simulink model "FOCsimulation"  (R2023b)
settings: Solver=VariableStepAuto  StartTime=0.0  StopTime=12  RelTol=1e-3
values from neighbouring files (symbols this model uses):
  acceleration = 20000/PU_System.N_base    [FOC_Script.m]    (also in Motor_script.m)
  PI_params = mcb.internal.SetControllerParameters(pmsm,inverter,PU_System,T_pwm,2*Ts,Ts_speed)    [FOC_Script.m]    (also in Motor_script.m)
  Speed_openLoop_PU = 0.1    [FOC_Script.m]    (also in Motor_script.m)
  T_Ref_openLoop = 1    [FOC_Script.m]    (also in Motor_script.m)
  Ts = T_pwm    (= 0.0001)    [FOC_Script.m]    (also in Motor_script.m = 3.33333333333e-05)
  Ts_motor = T_pwm/2    (= 5e-05)    [FOC_Script.m]    (also in Motor_script.m = 1.66666666667e-05)
  Ts_speed = 30*Ts    (= 0.003)    [FOC_Script.m]    (also in Motor_script.m = 0.001)
undefined symbols (not defined in the file or in its folder): inverter, pmsm, PU_System, sigbuilder_block, target
libraries: mcbcontrolslib x11, slpidlib x3, mcbpositiondecoderlib x2, simulink x1, dspsrcs4 x1, mcbplantlib x1, autolibpmsmexterior x1
(part 1 of 2)
settings Model: Creator=Juan Camilo  LastModifiedBy=84339
settings DebuggingCC: UnconnectedInputMsg=warning  UnconnectedOutputMsg=warning  UnconnectedLineMsg=warning
settings ModelReferenceCC: EnableRefExpFcnMdlSchedulingChecks=on
settings RTWCC: DLArmComputeVersion=19.05

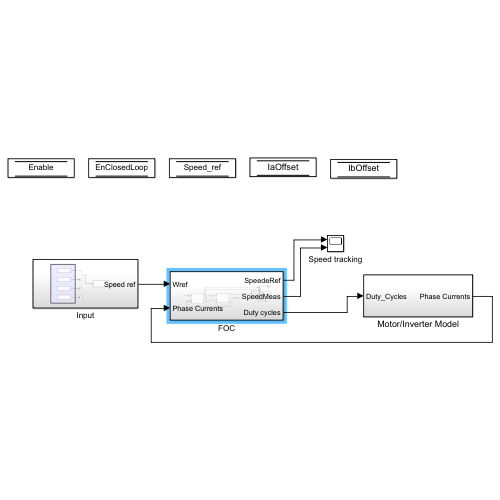
[thumbnail: Simulink's stored preview of the top-level diagram]
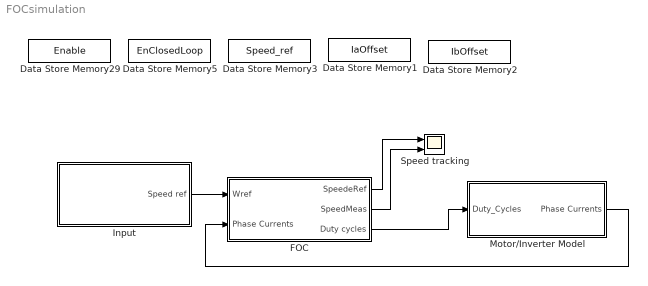
== system FOCsimulation ==
  Data Store Memory1 : DataStoreMemory  DataStoreName=IaOffset  InitialValue=inverter.CtSensAOffset  ShowAdditionalParam=off
  Data Store Memory2 : DataStoreMemory  DataStoreName=IbOffset  InitialValue=inverter.CtSensBOffset  ShowAdditionalParam=off
  Data Store Memory29 : DataStoreMemory  DataStoreName=Enable  ReadBeforeWriteMsg=warning  WriteAfterWriteMsg=warning  WriteAfterReadMsg=warning  ShowAdditionalParam=off  OutDataTypeStr=boolean
  Data Store Memory3 : DataStoreMemory  DataStoreName=Speed_ref  ReadBeforeWriteMsg=warning  WriteAfterWriteMsg=warning  WriteAfterReadMsg=warning  InitialValue=0.1  ShowAdditionalParam=off  OutDataTypeStr=dataType
  Data Store Memory5 : DataStoreMemory  DataStoreName=EnClosedLoop  ReadBeforeWriteMsg=warning  WriteAfterWriteMsg=warning  WriteAfterReadMsg=warning  ShowAdditionalParam=off  OutDataTypeStr=boolean
  FOC : Subsystem
  Input : Subsystem
  Motor/Inverter Model : Subsystem
  Speed tracking : Scope  NumInputPorts=2
  wires:
  Motor/Inverter Model/1(Phase Currents) -> FOC/2(Phase Currents)
  FOC/3(Duty cycles) -> Motor/Inverter Model/1(Duty_Cycles)
  Input/1(Speed ref) -> FOC/1(Wref)
  FOC/1(SpeedeRef) -> Speed tracking/1
  FOC/2(SpeedMeas) -> Speed tracking/2

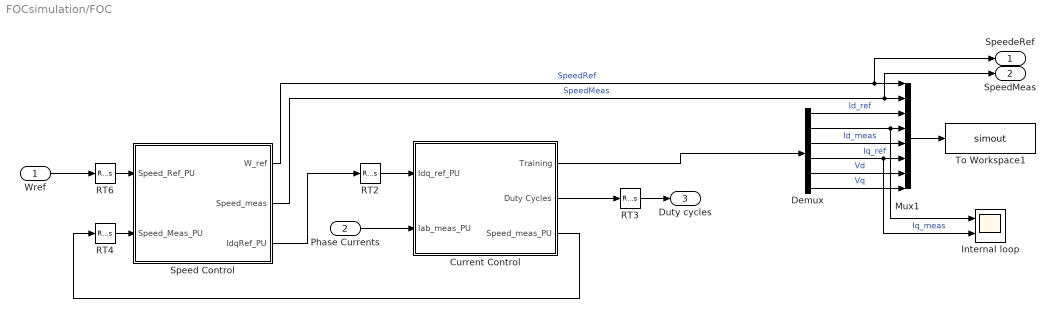
== system FOCsimulation/FOC ==
  Wref : Inport
  Phase Currents : Inport  Port=2
  Current Control : Subsystem
  Demux : Demux  Outputs=6
  Internal loop : Scope  NumInputPorts=2
  Mux1 : Mux  Inputs=8
  RT2 : RateTransition  Deterministic=off
  RT3 : RateTransition  Deterministic=off
  RT4 : RateTransition  Deterministic=off  OutPortSampleTime=Ts_speed
  RT6 : RateTransition  Deterministic=off  OutPortSampleTime=Ts_speed
  Speed Control : Subsystem  TreatAsAtomicUnit=on  SystemSampleTime=Ts_speed
  To Workspace1 : ToWorkspace  VariableName=simout  SaveFormat=Structure  SampleTime=-1
  SpeedeRef : Outport
  SpeedMeas : Outport  Port=2
  Duty cycles : Outport  Port=3
  wires:
  Speed Control/3(IdqRef_PU) -> RT2/1
  RT4/1 -> Speed Control/2(Speed_Meas_PU)
  RT2/1 -> Current Control/1(Idq_ref_PU)
  RT6/1 -> Speed Control/1(Speed_Ref_PU)
  Current Control/2(Duty Cycles) -> RT3/1
  RT3/1 -> Duty cycles/1
  Wref/1 -> RT6/1
  Phase Currents/1 -> Current Control/2(Iab_meas_PU)
  Current Control/3(Speed_meas_PU) -> RT4/1
  Mux1/1 -> To Workspace1/1
  Demux/1 -> Mux1/3  "Id_ref"
  Demux/2 -> Internal loop/1, Mux1/4  "Iq_ref"
  Demux/3 -> Mux1/5  "Id_meas"
  Demux/6 -> Mux1/8  "Vq"
  Demux/5 -> Mux1/7  "Vd"
  Current Control/1(Training) -> Demux/1
  Speed Control/2(Speed_meas) -> SpeedMeas/1, Mux1/2  "SpeedMeas"
  Speed Control/1(W_ref) -> SpeedeRef/1, Mux1/1  "SpeedRef"
  Demux/4 -> Mux1/6, Internal loop/2  "Iq_meas"

== system FOCsimulation/Input ==
  note: Input shapes
  Generated Signal : Subsystem
  Input Conditioning : Subsystem  SystemSampleTime=1e-3
  Ramp [Ts=10s] : Subsystem
  Random Signal [Ts=20s] : Subsystem
  Step [Ts=10s] : Subsystem
  Terminator : Terminator
  Terminator1 : Terminator
  Terminator2 : Terminator
  Speed ref : Outport
  wires:
  Input Conditioning/1(Desired Speed) -> Speed ref/1
  Generated Signal/1(Out1) -> Terminator/1
  Random Signal [Ts=20s]/1(Speed_Reference) -> Terminator1/1
  Ramp [Ts=10s]/1(Out1) -> Terminator2/1
  Step [Ts=10s]/1(Speed ref) -> Input Conditioning/1(Speed ref)

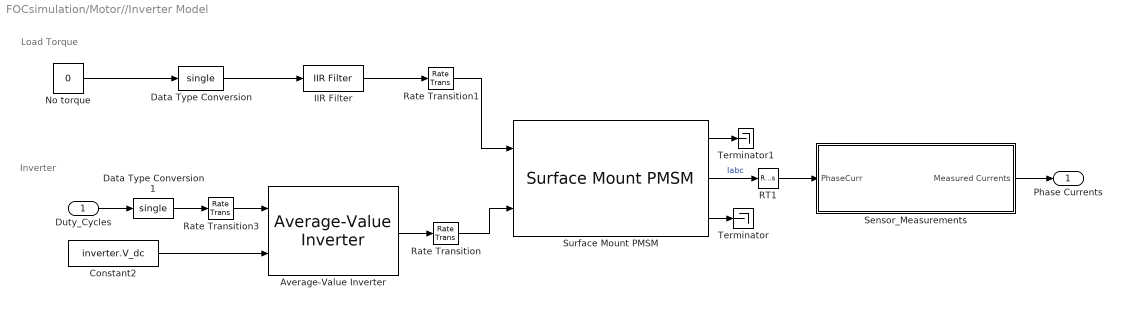
== system FOCsimulation/Motor//Inverter Model ==
  note: Load Torque
  note: Inverter
  Duty_Cycles : Inport
  Average-Value Inverter : mcbplantlib/Average-Value Inverter
  Constant2 : Constant  Value=inverter.V_dc  OutDataTypeStr=single  SampleTime=-1
  Data Type Conversion : DataTypeConversion  OutDataTypeStr=single  SaturateOnIntegerOverflow=off  RndMeth=Floor
  Data Type Conversion1 : DataTypeConversion  OutDataTypeStr=single  RndMeth=Simplest  SaturateOnIntegerOverflow=off
  IIR Filter : mcbcontrolslib/IIR Filter  VariantControl=Low Pass Filter  VariantSelect=Low-pass  Filter_constant=0.0001  advancedSettings=off  Ts=50e-6  cutOff_freq=0.31834
  No torque : Constant  Value=0
  RT1 : RateTransition  Deterministic=off  OutPortSampleTime=Ts_simulink
  Rate Transition : RateTransition  Deterministic=off  OutPortSampleTime=Ts_motor
  Rate Transition1 : RateTransition  Deterministic=off  OutPortSampleTime=Ts_motor
  Rate Transition3 : RateTransition  Deterministic=off  OutPortSampleTime=Ts_inverter
  Sensor_Measurements : Subsystem
  Surface Mount PMSM : autolibpmsmexterior/Surface Mount PMSM  port_config=Torque  sim_type=Discrete  Ts=Ts_motor  P=pmsm.p  Rs=pmsm.Rs + inverter.R_board  Ldq_=pmsm.Ld  KConstText=Permanent flux linkage constant (lambda_pm):  lambda_pm=pmsm.FluxPM  Ke=159.9771  Kt=1.323  mechanical=[pmsm.J, pmsm.B, 0]  idq0=[0 0]  theta_init=0  omega_init=0  KConst=pmsm.FluxPM  lambda_pm_calc=pmsm.FluxPM  RefBlkName='autolibpmsmexterior/Surface Mount PMSM'  aMode=5  Ldq="[0.0002      0.0002]"
  Terminator : Terminator
  Terminator1 : Terminator
  Phase Currents : Outport  VectorParamsAs1DForOutWhenUnconnected=off
  wires:
  Rate Transition1/1 -> Surface Mount PMSM/1
  IIR Filter/1 -> Rate Transition1/1
  Surface Mount PMSM/3 -> Terminator/1
  RT1/1 -> Sensor_Measurements/1(PhaseCurr)
  Surface Mount PMSM/2 -> RT1/1  "Iabc"
  Rate Transition/1 -> Surface Mount PMSM/2
  Duty_Cycles/1 -> Data Type Conversion1/1
  Data Type Conversion/1 -> IIR Filter/1
  Data Type Conversion1/1 -> Rate Transition3/1
  Rate Transition3/1 -> Average-Value Inverter/1
  Average-Value Inverter/1 -> Rate Transition/1
  Constant2/1 -> Average-Value Inverter/2
  No torque/1 -> Data Type Conversion/1
  Sensor_Measurements/1(Measured Currents) -> Phase Currents/1
  Surface Mount PMSM/1 -> Terminator1/1

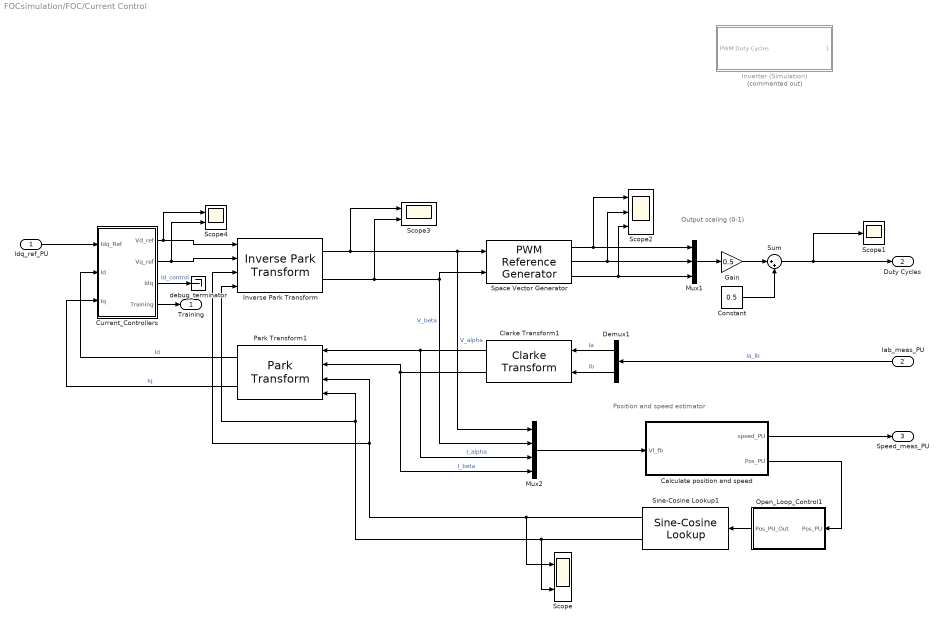
== system FOCsimulation/FOC/Current Control ==
  note: Position and speed estimator
  note: Output scaling (0-1)
  Idq_ref_PU : Inport
  Iab_meas_PU : Inport  Port=2
  Calculate position and speed : Subsystem
  Clarke Transform1 : mcbcontrolslib/Clarke Transform  VariantControl=Variant2  PhaseInput=Two inputs  EnPowerInv=off
  Constant : Constant  Value=0.5  OutDataTypeStr=dataType
  Current_Controllers : Subsystem
  Demux1 : Demux  Outputs=2
  Gain : Gain  Gain=0.5  OutDataTypeStr=Inherit: Same as input
  Inverse Park Transform : mcbcontrolslib/Inverse Park Transform  PhaseInput=Two inputs  AxisAlignment=D-axis  ThetaInput=Sine and Cosine electrical position  AngleInput=Per-unit  N_points=1024
  Inverter (Simulation) : Subsystem  Commented=on
  Mux1 : Mux  Inputs=3
  Mux2 : Mux
  Open_Loop_Control1 : Subsystem
  Park Transform1 : mcbcontrolslib/Park Transform  PhaseInput=Two inputs  AxisAlignment=D-axis  ThetaInput=Sine and Cosine electrical position  AngleInput=Per-unit  N_points=1024
  Scope : Scope  NumInputPorts=2
  Scope1 : Scope
  Scope2 : Scope  NumInputPorts=3
  Scope3 : Scope  NumInputPorts=2
  Scope4 : Scope  NumInputPorts=2
  Sine-Cosine Lookup1 : mcbcontrolslib/Sine-Cosine Lookup  AngleInput=Per-unit  N_points=1024
  Space Vector Generator : mcbcontrolslib/PWM Reference Generator  inSignal=Valphabeta  modType=SVM: space vector modulation
  Sum : Sum  Inputs=|++
  debug_terminator : Terminator
  Training : Outport  VectorParamsAs1DForOutWhenUnconnected=off
  Duty Cycles : Outport  Port=2  VectorParamsAs1DForOutWhenUnconnected=off
  Speed_meas_PU : Outport  Port=3  InitialOutput=0  VectorParamsAs1DForOutWhenUnconnected=off
  wires:
  Current_Controllers/1(Vd_ref) -> Scope4/1, Inverse Park Transform/1
  Inverse Park Transform/2 -> Scope3/2, Space Vector Generator/2, Mux2/2  "V_beta"
  Inverse Park Transform/1 -> Scope3/1, Space Vector Generator/1, Mux2/1  "V_alpha"
  Mux2/1 -> Calculate position and speed/1(VI_fb)
  Current_Controllers/2(Vq_ref) -> Scope4/2, Inverse Park Transform/2
  Space Vector Generator/1 -> Scope2/1, Mux1/1
  Space Vector Generator/3 -> Mux1/3, Scope2/3
  Space Vector Generator/2 -> Scope2/2, Mux1/2
  Idq_ref_PU/1 -> Current_Controllers/1(Idq_Ref)
  Current_Controllers/3(Idq) -> debug_terminator/1  "Id_control"
  Mux1/1 -> Gain/1
  Gain/1 -> Sum/1
  Constant/1 -> Sum/2
  Calculate position and speed/1(speed_PU) -> Speed_meas_PU/1
  Clarke Transform1/1 -> Mux2/3, Park Transform1/1  "I_alpha"
  Clarke Transform1/2 -> Mux2/4, Park Transform1/2  "I_beta"
  Sine-Cosine Lookup1/1 -> Scope/1, Park Transform1/3, Inverse Park Transform/3
  Sine-Cosine Lookup1/2 -> Scope/2, Park Transform1/4, Inverse Park Transform/4
  Demux1/1 -> Clarke Transform1/1  "Ia"
  Demux1/2 -> Clarke Transform1/2  "Ib"
  Open_Loop_Control1/1(Pos_PU_Out) -> Sine-Cosine Lookup1/1
  Iab_meas_PU/1 -> Demux1/1  "Ia_Ib"
  Park Transform1/1 -> Current_Controllers/2(Id)  "Id"
  Park Transform1/2 -> Current_Controllers/3(Iq)  "Iq"
  Calculate position and speed/2(Pos_PU) -> Open_Loop_Control1/1(Pos_PU)
  Current_Controllers/4(Training) -> Training/1
  Sum/1 -> Scope1/1, Duty Cycles/1

== system FOCsimulation/FOC/Speed Control ==
  Speed_Ref_PU : Inport
  Speed_Meas_PU : Inport  Port=2
  Id_Ref : Constant  Value=0  OutDataTypeStr=dataType
  Mux : Mux  Inputs=2
  PI_Controller_Speed : Subsystem
  Speed_Ref_Selector : Subsystem
  W_ref : Outport  VectorParamsAs1DForOutWhenUnconnected=off
  Speed_meas : Outport  Port=2  VectorParamsAs1DForOutWhenUnconnected=off
  IdqRef_PU : Outport  Port=3  VectorParamsAs1DForOutWhenUnconnected=off
  wires:
  PI_Controller_Speed/1(Iq_ref) -> Mux/2
  Speed_Meas_PU/1 -> PI_Controller_Speed/2(N_fb)  "Speed_fb"
  Id_Ref/1 -> Mux/1
  Mux/1 -> IdqRef_PU/1
  Speed_Ref_Selector/1(Speed_Ref1) -> PI_Controller_Speed/1(N_ref)  "Speed_ref"
  Speed_Ref_PU/1 -> Speed_Ref_Selector/1(Speed_Ref)
  PI_Controller_Speed/2(W_ref) -> W_ref/1
  PI_Controller_Speed/3(Speed_meas) -> Speed_meas/1

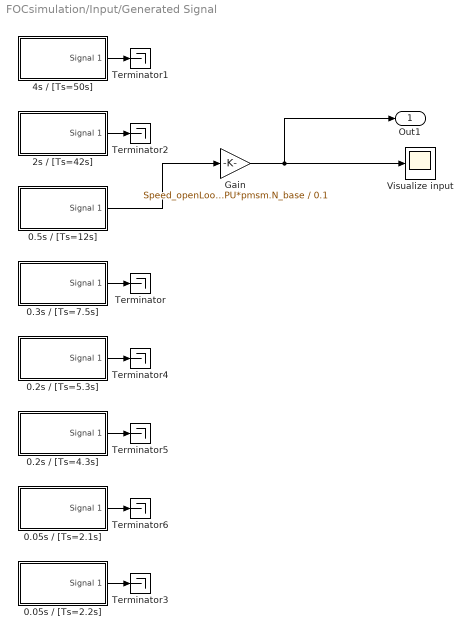
== system FOCsimulation/Input/Generated Signal ==
  0.05s / [Ts=2.1s] : Subsystem  Tag=STV Subsys  LoadFcn=sigbuilder_block('load');  StartFcn=sigbuilder_block('start');  StopFcn=sigbuilder_block('stop');  ClipboardFcn=sigbuilder_block('clipboard');  mask(Sigbuilder block){tuvar=[0:10]}
      mask help: Simulink:masks:SigbuilderBlock_MD
      mask init:
      | if ~strcmp(get_param(bdroot(gcbh),'SimulationStatus'),'stopped') tuvar = sigbuilder_block('maskInit'); end
      settings: CopyFcn=sigbuilder_block('copy');  DeleteFcn=sigbuilder_block('delete');  ModelCloseFcn=sigbuilder_block('modelClose');  PreSaveFcn=sigbuilder_block('preSave');  PauseFcn=sigbuilder_block('pause');  ContinueFcn=sigbuilder_block('continue');  NameChangeFcn=sigbuilder_block('namechange');  OpenFcn=sigbuilder_block('open',[5.4 5.4 1141.2 580.8 ]);  CloseFcn=sigbuilder_block('close');
      mask Display: plot(0, 0, 100, 100,[2, 2, 32, 32, 2], [68, 8, 8, 68, 68],[32, 2], [38, 38], [32, 19, 2],[53, 60, 44], [32, 17, 17, 2],[16, 16, 31, 31]);txt = getActiveGroup(gcbh);text(2, 100, txt,'verticalAlignment', 'top');
  0.05s / [Ts=2.2s] : Subsystem  Tag=STV Subsys  LoadFcn=sigbuilder_block('load');  StartFcn=sigbuilder_block('start');  StopFcn=sigbuilder_block('stop');  ClipboardFcn=sigbuilder_block('clipboard');  mask(Sigbuilder block){tuvar=[0:10]}
      mask help: Simulink:masks:SigbuilderBlock_MD
      mask init:
      | if ~strcmp(get_param(bdroot(gcbh),'SimulationStatus'),'stopped') tuvar = sigbuilder_block('maskInit'); end
      settings: CopyFcn=sigbuilder_block('copy');  DeleteFcn=sigbuilder_block('delete');  ModelCloseFcn=sigbuilder_block('modelClose');  PreSaveFcn=sigbuilder_block('preSave');  PauseFcn=sigbuilder_block('pause');  ContinueFcn=sigbuilder_block('continue');  NameChangeFcn=sigbuilder_block('namechange');  OpenFcn=sigbuilder_block('open',[5.4 5.4 1141.2 580.8 ]);  CloseFcn=sigbuilder_block('close');
      mask Display: plot(0, 0, 100, 100,[2, 2, 32, 32, 2], [68, 8, 8, 68, 68],[32, 2], [38, 38], [32, 19, 2],[53, 60, 44], [32, 17, 17, 2],[16, 16, 31, 31]);txt = getActiveGroup(gcbh);text(2, 100, txt,'verticalAlignment', 'top');
  0.2s / [Ts=4.3s] : Subsystem  Tag=STV Subsys  LoadFcn=sigbuilder_block('load');  StartFcn=sigbuilder_block('start');  StopFcn=sigbuilder_block('stop');  ClipboardFcn=sigbuilder_block('clipboard');  mask(Sigbuilder block){tuvar=[0:10]}
      mask help: Simulink:masks:SigbuilderBlock_MD
      mask init:
      | if ~strcmp(get_param(bdroot(gcbh),'SimulationStatus'),'stopped') tuvar = sigbuilder_block('maskInit'); end
      settings: CopyFcn=sigbuilder_block('copy');  DeleteFcn=sigbuilder_block('delete');  ModelCloseFcn=sigbuilder_block('modelClose');  PreSaveFcn=sigbuilder_block('preSave');  PauseFcn=sigbuilder_block('pause');  ContinueFcn=sigbuilder_block('continue');  NameChangeFcn=sigbuilder_block('namechange');  OpenFcn=sigbuilder_block('open',[5.4 5.4 1141.2 580.8 ]);  CloseFcn=sigbuilder_block('close');
      mask Display: plot(0, 0, 100, 100,[2, 2, 32, 32, 2], [68, 8, 8, 68, 68],[32, 2], [38, 38], [32, 19, 2],[53, 60, 44], [32, 17, 17, 2],[16, 16, 31, 31]);txt = getActiveGroup(gcbh);text(2, 100, txt,'verticalAlignment', 'top');
  0.2s / [Ts=5.3s] : Subsystem  Tag=STV Subsys  LoadFcn=sigbuilder_block('load');  StartFcn=sigbuilder_block('start');  StopFcn=sigbuilder_block('stop');  ClipboardFcn=sigbuilder_block('clipboard');  mask(Sigbuilder block){tuvar=[0:10]}
      mask help: Simulink:masks:SigbuilderBlock_MD
      mask init:
      | if ~strcmp(get_param(bdroot(gcbh),'SimulationStatus'),'stopped') tuvar = sigbuilder_block('maskInit'); end
      settings: CopyFcn=sigbuilder_block('copy');  DeleteFcn=sigbuilder_block('delete');  ModelCloseFcn=sigbuilder_block('modelClose');  PreSaveFcn=sigbuilder_block('preSave');  PauseFcn=sigbuilder_block('pause');  ContinueFcn=sigbuilder_block('continue');  NameChangeFcn=sigbuilder_block('namechange');  OpenFcn=sigbuilder_block('open',[1440 -126 1440 717.6 ]);  CloseFcn=sigbuilder_block('close');
      mask Display: plot(0, 0, 100, 100,[2, 2, 32, 32, 2], [68, 8, 8, 68, 68],[32, 2], [38, 38], [32, 19, 2],[53, 60, 44], [32, 17, 17, 2],[16, 16, 31, 31]);txt = getActiveGroup(gcbh);text(2, 100, txt,'verticalAlignment', 'top');
  0.3s / [Ts=7.5s] : Subsystem  Tag=STV Subsys  LoadFcn=sigbuilder_block('load');  StartFcn=sigbuilder_block('start');  StopFcn=sigbuilder_block('stop');  ClipboardFcn=sigbuilder_block('clipboard');  mask(Sigbuilder block){tuvar=[0:10]}
      mask help: Simulink:masks:SigbuilderBlock_MD
      mask init:
      | if ~strcmp(get_param(bdroot(gcbh),'SimulationStatus'),'stopped') tuvar = sigbuilder_block('maskInit'); end
      settings: CopyFcn=sigbuilder_block('copy');  DeleteFcn=sigbuilder_block('delete');  ModelCloseFcn=sigbuilder_block('modelClose');  PreSaveFcn=sigbuilder_block('preSave');  PauseFcn=sigbuilder_block('pause');  ContinueFcn=sigbuilder_block('continue');  NameChangeFcn=sigbuilder_block('namechange');  OpenFcn=sigbuilder_block('open',[5.4 36 1141.2 516.6 ]);  CloseFcn=sigbuilder_block('close');
      mask Display: plot(0, 0, 100, 100,[2, 2, 32, 32, 2], [68, 8, 8, 68, 68],[32, 2], [38, 38], [32, 19, 2],[53, 60, 44], [32, 17, 17, 2],[16, 16, 31, 31]);txt = getActiveGroup(gcbh);text(2, 100, txt,'verticalAlignment', 'top');
  0.5s / [Ts=12s] : Subsystem  Tag=STV Subsys  LoadFcn=sigbuilder_block('load');  StartFcn=sigbuilder_block('start');  StopFcn=sigbuilder_block('stop');  ClipboardFcn=sigbuilder_block('clipboard');  mask(Sigbuilder block){tuvar=[0:10]}
      mask help: Simulink:masks:SigbuilderBlock_MD
      mask init:
      | if ~strcmp(get_param(bdroot(gcbh),'SimulationStatus'),'stopped') tuvar = sigbuilder_block('maskInit'); end
      settings: CopyFcn=sigbuilder_block('copy');  DeleteFcn=sigbuilder_block('delete');  ModelCloseFcn=sigbuilder_block('modelClose');  PreSaveFcn=sigbuilder_block('preSave');  PauseFcn=sigbuilder_block('pause');  ContinueFcn=sigbuilder_block('continue');  NameChangeFcn=sigbuilder_block('namechange');  OpenFcn=sigbuilder_block('open',[5.4 36 1141.2 516.6 ]);  CloseFcn=sigbuilder_block('close');
      mask Display: plot(0, 0, 100, 100,[2, 2, 32, 32, 2], [68, 8, 8, 68, 68],[32, 2], [38, 38], [32, 19, 2],[53, 60, 44], [32, 17, 17, 2],[16, 16, 31, 31]);txt = getActiveGroup(gcbh);text(2, 100, txt,'verticalAlignment', 'top');
  2s / [Ts=42s] : Subsystem  Tag=STV Subsys  LoadFcn=sigbuilder_block('load');  StartFcn=sigbuilder_block('start');  StopFcn=sigbuilder_block('stop');  ClipboardFcn=sigbuilder_block('clipboard');  mask(Sigbuilder block){tuvar=[0:10]}
      mask help: Simulink:masks:SigbuilderBlock_MD
      mask init:
      | if ~strcmp(get_param(bdroot(gcbh),'SimulationStatus'),'stopped') tuvar = sigbuilder_block('maskInit'); end
      settings: CopyFcn=sigbuilder_block('copy');  DeleteFcn=sigbuilder_block('delete');  ModelCloseFcn=sigbuilder_block('modelClose');  PreSaveFcn=sigbuilder_block('preSave');  PauseFcn=sigbuilder_block('pause');  ContinueFcn=sigbuilder_block('continue');  NameChangeFcn=sigbuilder_block('namechange');  OpenFcn=sigbuilder_block('open',[5.4 36.6 1141.2 516.6 ]);  CloseFcn=sigbuilder_block('close');
      mask Display: plot(0, 0, 100, 100,[2, 2, 32, 32, 2], [68, 8, 8, 68, 68],[32, 2], [38, 38], [32, 19, 2],[53, 60, 44], [32, 17, 17, 2],[16, 16, 31, 31]);txt = getActiveGroup(gcbh);text(2, 100, txt,'verticalAlignment', 'top');
  4s / [Ts=50s] : Subsystem  Tag=STV Subsys  LoadFcn=sigbuilder_block('load');  StartFcn=sigbuilder_block('start');  StopFcn=sigbuilder_block('stop');  ClipboardFcn=sigbuilder_block('clipboard');  mask(Sigbuilder block){tuvar=[0:10]}
      mask help: Simulink:masks:SigbuilderBlock_MD
      mask init:
      | if ~strcmp(get_param(bdroot(gcbh),'SimulationStatus'),'stopped') tuvar = sigbuilder_block('maskInit'); end
      settings: CopyFcn=sigbuilder_block('copy');  DeleteFcn=sigbuilder_block('delete');  ModelCloseFcn=sigbuilder_block('modelClose');  PreSaveFcn=sigbuilder_block('preSave');  PauseFcn=sigbuilder_block('pause');  ContinueFcn=sigbuilder_block('continue');  NameChangeFcn=sigbuilder_block('namechange');  OpenFcn=sigbuilder_block('open',[0.6 36.6 574.8 494.4 ]);  CloseFcn=sigbuilder_block('close');
      mask Display: plot(0, 0, 100, 100,[2, 2, 32, 32, 2], [68, 8, 8, 68, 68],[32, 2], [38, 38], [32, 19, 2],[53, 60, 44], [32, 17, 17, 2],[16, 16, 31, 31]);txt = getActiveGroup(gcbh);text(2, 100, txt,'verticalAlignment', 'top');
  Gain : Gain  Gain=Speed_openLoop_PU*pmsm.N_base / 0.1
  Terminator{,1..6} (7 alike) : Terminator
  Visualize input : Scope
  Out1 : Outport
  wires:
  Gain/1 -> Out1/1, Visualize input/1
  4s / [Ts=50s]/1(Signal 1) -> Terminator1/1
  2s / [Ts=42s]/1(Signal 1) -> Terminator2/1
  0.3s / [Ts=7.5s]/1(Signal 1) -> Terminator/1
  0.2s / [Ts=5.3s]/1(Signal 1) -> Terminator4/1
  0.2s / [Ts=4.3s]/1(Signal 1) -> Terminator5/1
  0.05s / [Ts=2.1s]/1(Signal 1) -> Terminator6/1
  0.5s / [Ts=12s]/1(Signal 1) -> Gain/1
  0.05s / [Ts=2.2s]/1(Signal 1) -> Terminator3/1

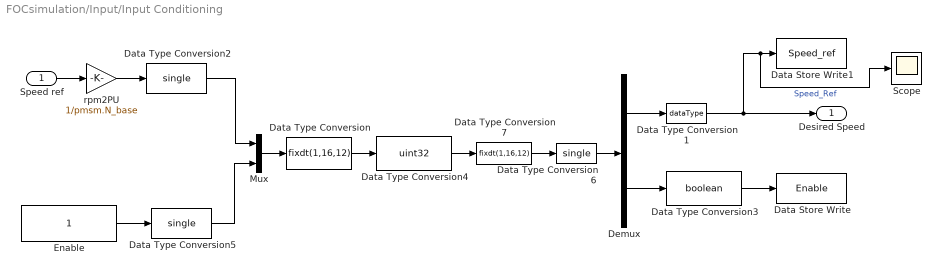
== system FOCsimulation/Input/Input Conditioning ==
  Speed ref : Inport
  Data Store Write : DataStoreWrite  DataStoreName=Enable  IndexOptions=Index vector (dialog)  Indices=1  OutputSizes=1
  Data Store Write1 : DataStoreWrite  DataStoreName=Speed_ref  IndexOptions=Index vector (dialog)  Indices=1  OutputSizes=1
  Data Type Conversion : DataTypeConversion  OutDataTypeStr=fixdt(1,16,12)  RndMeth=Simplest  SaturateOnIntegerOverflow=off
  Data Type Conversion1 : DataTypeConversion  OutDataTypeStr=dataType  RndMeth=Simplest  SaturateOnIntegerOverflow=off
  Data Type Conversion2 : DataTypeConversion  OutDataTypeStr=single  RndMeth=Simplest  SaturateOnIntegerOverflow=off
  Data Type Conversion3 : DataTypeConversion  OutDataTypeStr=boolean  RndMeth=Simplest  SaturateOnIntegerOverflow=off
  Data Type Conversion4 : DataTypeConversion  OutDataTypeStr=uint32  ConvertRealWorld=Stored Integer (SI)  RndMeth=Simplest  SaturateOnIntegerOverflow=off
  Data Type Conversion5 : DataTypeConversion  OutDataTypeStr=single  RndMeth=Simplest  SaturateOnIntegerOverflow=off
  Data Type Conversion6 : DataTypeConversion  OutDataTypeStr=single  RndMeth=Simplest  SaturateOnIntegerOverflow=off
  Data Type Conversion7 : DataTypeConversion  OutDataTypeStr=fixdt(1,16,12)  ConvertRealWorld=Stored Integer (SI)  RndMeth=Simplest  SaturateOnIntegerOverflow=off
  Demux : Demux  Outputs=2
  Enable : Constant  OutDataTypeStr=dataType  SampleTime=-1
  Mux : Mux  Inputs=2
  Scope : Scope
  rpm2PU : Gain  Gain=1/pmsm.N_base  RndMeth=Simplest  OutDataTypeStr=Inherit: Same as input
  Desired Speed : Outport  VectorParamsAs1DForOutWhenUnconnected=off
  wires:
  Data Type Conversion1/1 -> Scope/1, Data Store Write1/1, Desired Speed/1  "Speed_Ref"
  Demux/1 -> Data Type Conversion1/1
  Data Type Conversion3/1 -> Data Store Write/1
  Demux/2 -> Data Type Conversion3/1
  Mux/1 -> Data Type Conversion/1
  Enable/1 -> Data Type Conversion5/1
  rpm2PU/1 -> Data Type Conversion2/1
  Data Type Conversion5/1 -> Mux/2
  Data Type Conversion/1 -> Data Type Conversion4/1
  Data Type Conversion2/1 -> Mux/1
  Speed ref/1 -> rpm2PU/1
  Data Type Conversion7/1 -> Data Type Conversion6/1
  Data Type Conversion6/1 -> Demux/1
  Data Type Conversion4/1 -> Data Type Conversion7/1

== system FOCsimulation/Input/Ramp [Ts=10s] ==
  note: Delay Random signal
  Constant : Constant  Value=0
  Enable : Step  Time=T_Ref_openLoop
  OpenLoop Start : Step  Time=T_Ref_openLoop  Before=Speed_openLoop_PU*pmsm.N_base  After=0
  Ramp from base speed : simulink/Sources/Ramp  slope=pmsm.N_base*0.8  start=T_Ref_openLoop  InitialOutput=Speed_openLoop_PU*pmsm.N_base + 1
  Sum : Sum  Inputs=|++
  Switch1 : Switch  Threshold=0.5  RndMeth=Simplest  SaturateOnIntegerOverflow=off  InputSameDT=off
  Out1 : Outport
  wires:
  Ramp from base speed/1 -> Switch1/1
  Enable/1 -> Switch1/2
  Switch1/1 -> Sum/2
  Constant/1 -> Switch1/3
  OpenLoop Start/1 -> Sum/1
  Sum/1 -> Out1/1

== system FOCsimulation/Input/Random Signal [Ts=20s] ==
  note: Delay Random signal
  Constant : Constant  Value=0
  Enable : Step  Time=T_Ref_openLoop
  Gain : Gain  Gain=100
  OpenLoop Start : Step  Time=T_Ref_openLoop  Before=Speed_openLoop_PU*pmsm.N_base  After=Speed_openLoop_PU*pmsm.N_base
  Random Source : dspsrcs4/Random Source  SrcType=Uniform  NormMethod=Ziggurat  CltLength=12  MinVal=30  MaxVal=35  MeanVal=0  VarVal=1  RepMode=Repeatable  rawSeed=1  IsInherit=on  SampMode=Continuous  SampTime=-1  SampFrame=1  DataType=Double  OutComplex=Real  OutputFrames=off
  Sum : Sum  Inputs=|++
  Switch1 : Switch  Threshold=0.5  RndMeth=Simplest  SaturateOnIntegerOverflow=off  InputSameDT=off
  Speed_Reference : Outport
  wires:
  OpenLoop Start/1 -> Sum/1
  Sum/1 -> Speed_Reference/1
  Switch1/1 -> Sum/2
  Enable/1 -> Switch1/2
  Constant/1 -> Switch1/3
  Gain/1 -> Switch1/1
  Random Source/1 -> Gain/1

== system FOCsimulation/Input/Step [Ts=10s] ==
  Speed_Ref_CW (rpm)1 : Step  Time=T_Ref_openLoop  Before=Speed_openLoop_PU*pmsm.N_base  After=0.4*pmsm.N_base
  Speed ref : Outport
  wires:
  Speed_Ref_CW (rpm)1/1 -> Speed ref/1

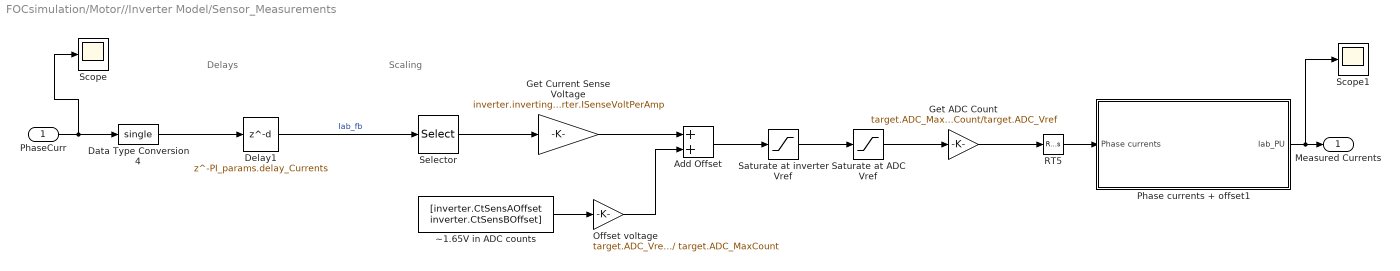
== system FOCsimulation/Motor//Inverter Model/Sensor_Measurements ==
  note: Scaling
  note: Delays
  PhaseCurr : Inport
  Add Offset : Sum  RndMeth=Simplest
  Data Type Conversion4 : DataTypeConversion  OutDataTypeStr=single  RndMeth=Simplest  SaturateOnIntegerOverflow=off
  Delay1 : Delay  DelayLength=PI_params.delay_Currents
  Get ADC Count : Gain  Gain=target.ADC_MaxCount/target.ADC_Vref  OutMin=0  OutMax=target.ADC_MaxCount  OutDataTypeStr=uint16  RndMeth=Simplest
  Get Current Sense Voltage : Gain  Gain=inverter.invertingAmp * inverter.ISenseVoltPerAmp  RndMeth=Simplest  OutDataTypeStr=Inherit: Same as input
  Offset voltage : Gain  Gain=target.ADC_Vref / target.ADC_MaxCount  RndMeth=Simplest
  Phase currents + offset1 : Subsystem
  RT5 : RateTransition  Deterministic=off
  Saturate at ADC Vref : Saturate  UpperLimit=target.ADC_Vref  LowerLimit=0
  Saturate at inverter Vref : Saturate  UpperLimit=inverter.ISenseVref  LowerLimit=0
  Scope : Scope
  Scope1 : Scope
  Selector : Selector  InputPortWidth=3  IndexOptions=Index vector (dialog)  Indices=[1 2]  OutputSizes=1
  ~1.65V in ADC counts : Constant  Value=[inverter.CtSensAOffset inverter.CtSensBOffset]  OutDataTypeStr=uint16  SampleTime=-1
  Measured Currents : Outport  VectorParamsAs1DForOutWhenUnconnected=off
  wires:
  Delay1/1 -> Selector/1  "Iab_fb"
  Data Type Conversion4/1 -> Delay1/1
  PhaseCurr/1 -> Scope/1, Data Type Conversion4/1
  Add Offset/1 -> Saturate at inverter Vref/1
  Saturate at inverter Vref/1 -> Saturate at ADC Vref/1
  ~1.65V in ADC counts/1 -> Offset voltage/1
  Get Current Sense Voltage/1 -> Add Offset/1
  Saturate at ADC Vref/1 -> Get ADC Count/1
  Selector/1 -> Get Current Sense Voltage/1
  Offset voltage/1 -> Add Offset/2
  Phase currents + offset1/1(Iab_PU) -> Scope1/1, Measured Currents/1
  Get ADC Count/1 -> RT5/1
  RT5/1 -> Phase currents + offset1/1(Phase currents)

== system FOCsimulation/FOC/Current Control/Calculate position and speed ==
  VI_fb : Inport
  Delay5 : Delay  DelayLength=1
  Demux : Demux  Outputs=2
  Flux Observer : Subsystem
  speed_PU : Outport
  Pos_PU : Outport  Port=2
  wires:
  VI_fb/1 -> Delay5/1
  Demux/1 -> Pos_PU/1
  Demux/2 -> speed_PU/1
  Flux Observer/1(Position/Speed) -> Demux/1
  Delay5/1 -> Flux Observer/1(InputSignals)

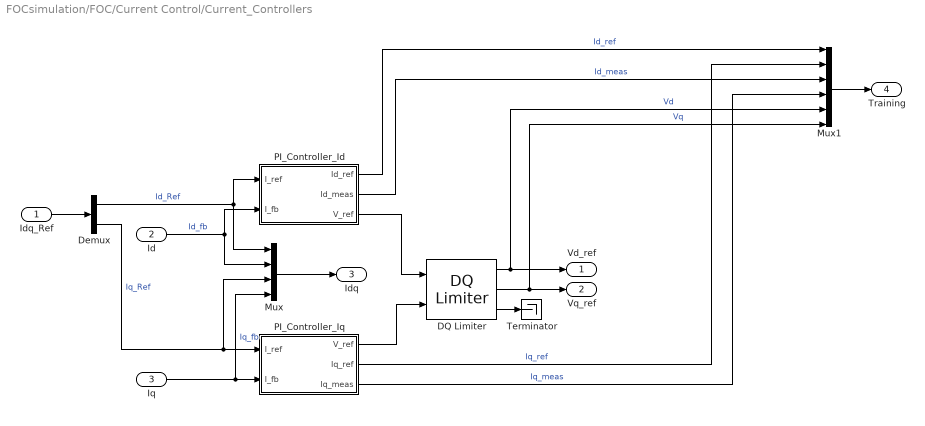
== system FOCsimulation/FOC/Current Control/Current_Controllers ==
  Idq_Ref : Inport
  Id : Inport  Port=2
  Iq : Inport  Port=3
  DQ Limiter : mcbcontrolslib/DQ Limiter  satMethodInputType=Specify via dialog  satMethodSelected=D-Q equivalence  satLimitInputType=Specify via dialog  Vmax=1
  Demux : Demux  Outputs=2
  Mux : Mux
  Mux1 : Mux  Inputs=6
  PI_Controller_Id : Subsystem
  PI_Controller_Iq : Subsystem
  Terminator : Terminator
  Vd_ref : Outport  VectorParamsAs1DForOutWhenUnconnected=off
  Vq_ref : Outport  Port=2  VectorParamsAs1DForOutWhenUnconnected=off
  Idq : Outport  Port=3  VectorParamsAs1DForOutWhenUnconnected=off
  Training : Outport  Port=4  VectorParamsAs1DForOutWhenUnconnected=off
  wires:
  Iq/1 -> Mux/4, PI_Controller_Iq/2(I_fb)  "Iq_fb"
  PI_Controller_Id/3(V_ref) -> DQ Limiter/1
  Id/1 -> PI_Controller_Id/2(I_fb), Mux/2  "Id_fb"
  Demux/1 -> PI_Controller_Id/1(I_ref), Mux/1  "Id_Ref"
  Demux/2 -> Mux/3, PI_Controller_Iq/1(I_ref)  "Iq_Ref"
  DQ Limiter/1 -> Mux1/5, Vd_ref/1  "Vd"
  DQ Limiter/2 -> Mux1/6, Vq_ref/1  "Vq"
  PI_Controller_Iq/1(V_ref) -> DQ Limiter/2
  DQ Limiter/3 -> Terminator/1
  Idq_Ref/1 -> Demux/1
  Mux/1 -> Idq/1
  Mux1/1 -> Training/1
  PI_Controller_Id/1(Id_ref) -> Mux1/1  "Id_ref"
  PI_Controller_Id/2(Id_meas) -> Mux1/3  "Id_meas"
  PI_Controller_Iq/2(Iq_ref) -> Mux1/2  "Iq_ref"
  PI_Controller_Iq/3(Iq_meas) -> Mux1/4  "Iq_meas"

== system FOCsimulation/FOC/Current Control/Inverter (Simulation) ==
  PWM Duty Cycles : Inport
  Data Type Duplicate : DataTypeDuplicate
  Data Type Conversion : DataTypeConversion  OutDataTypeStr=dataType  SaturateOnIntegerOverflow=off  RndMeth=Floor
  Enable : DataStoreRead  DataStoreName=Enable  IndexOptions=Index vector (dialog)  Indices=1  OutputSizes=1
  Mux2 : Mux  Inputs=3
  Switch1 : Switch  Threshold=0.5  RndMeth=Simplest  SaturateOnIntegerOverflow=off  InputSameDT=off
  stop : Constant  Value=0  OutDataTypeStr=Inherit: Inherit via back propagation
  " " : Outport  VectorParamsAs1DForOutWhenUnconnected=off
  wires:
  stop/1 -> Data Type Duplicate/2, Mux2/1, Mux2/3, Mux2/2
  Mux2/1 -> Switch1/3
  Switch1/1 -> " "/1
  Data Type Conversion/1 -> Switch1/2  "PWM Enable"
  PWM Duty Cycles/1 -> Data Type Duplicate/1, Switch1/1  "PWM Duty Cycles"
  Enable/1 -> Data Type Conversion/1

== system FOCsimulation/FOC/Current Control/Open_Loop_Control1 ==
  Pos_PU : Inport
  Abs : Abs  SaturateOnIntegerOverflow=off
  Constant : Constant  OutDataTypeStr=uint16
  Constant1 : Constant  Value=0  OutDataTypeStr=uint16
  Data Store Read : DataStoreRead  DataStoreName=Speed_ref  IndexOptions=Index vector (dialog)  Indices=1  OutputSizes=1
  Data Store Write : DataStoreWrite  DataStoreName=EnClosedLoop  IndexOptions=Index vector (dialog)  Indices=1  OutputSizes=1
  Data Type Conversion : DataTypeConversion  OutDataTypeStr=boolean  RndMeth=Simplest  SaturateOnIntegerOverflow=off
  Gain : Gain  Gain=Ts*PU_System.N_base*pmsm.p/60  OutDataTypeStr=Inherit: Same as input  ParamDataTypeStr=Inherit: Same as input
  Position Generator : mcbcontrolslib/Position Generator  AngleOutput=Per-unit  ExternalReset=none  Offset=0
  Switch : Switch  Criteria=u2 ~= 0  Threshold=0.1  SaturateOnIntegerOverflow=off  InputSameDT=off
  Switch2 : Switch  Criteria=u2 > Threshold  Threshold=Speed_openLoop_PU  SaturateOnIntegerOverflow=off  InputSameDT=off
  Pos_PU_Out : Outport
  wires:
  Constant1/1 -> Switch2/3
  Constant/1 -> Switch2/1
  Abs/1 -> Switch2/2
  Pos_PU/1 -> Switch/1
  Switch/1 -> Pos_PU_Out/1
  Gain/1 -> Position Generator/1
  Switch2/1 -> Switch/2, Data Type Conversion/1
  Data Store Read/1 -> Abs/1, Gain/1
  Data Type Conversion/1 -> Data Store Write/1
  Position Generator/1 -> Switch/3  "Pos_Open_Loop"

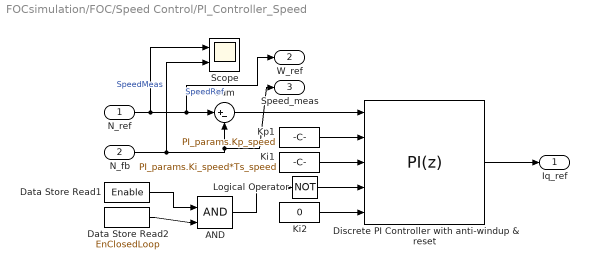
== system FOCsimulation/FOC/Speed Control/PI_Controller_Speed ==
  N_ref : Inport
  N_fb : Inport  Port=2
  AND : Logic  IconShape=distinctive  AllPortsSameDT=off  OutDataTypeStr=boolean
  Data Store Read2 : DataStoreRead  DataStoreName=EnClosedLoop  IndexOptions=Index vector (dialog)  Indices=1  OutputSizes=1
  Data Store Read1 : DataStoreRead  DataStoreName=Enable  IndexOptions=Index vector (dialog)  Indices=1  OutputSizes=1
  Discrete PI Controller with anti-windup & reset : slpidlib/PID Controller  Controller=PI  Form=Parallel  TimeDomain=Discrete-time  UseExternalTs=off  SampleTime=-1  IntegratorMethod=Forward Euler  FilterMethod=Forward Euler  ControllerParametersSource=external  P=1  I=1  UseKiTs=on  D=0  N=100  UseFilter=on  TunerSelectOption=Transfer Function Based (PID Tuner App)  InitialConditionSource=external  InitialConditionForIntegrator=0  InitialConditionForFilter=0  DifferentiatorICPrevScaledInput=0  ExternalReset=level  TrackingMode=off  Kt=1  LimitOutput=on  SatLimitsSource=internal  UpperSaturationLimit=1  LowerSaturationLimit=-1  LinearizeAsGain=on  AntiWindupMode=clamping  Kb=1  LimitIntegrator=off  UpperIntegratorSaturationLimit=inf  LowerIntegratorSaturationLimit=-inf  RndMeth=Simplest  POutMin=[]  POutMax=[]  IOutMin=[]  IOutMax=[]  DOutMin=[]  DOutMax=[]  NOutMin=[]  NOutMax=[]  SumOutMin=[]  SumOutMax=[]  SaturationOutDataTypeStr=Inherit: Inherit via back propagation  SaturationOutMin=[]  SaturationOutMax=[]  PParamMin=[]  PParamMax=[]  IParamMin=[]  IParamMax=[]  DParamMin=[]  DParamMax=[]  NParamMin=[]  NParamMax=[]  KbParamMin=[]  KbParamMax=[]  KtParamMin=[]  KtParamMax=[]  KbOutMin=[]  KbOutMax=[]  KtOutMin=[]  KtOutMax=[]  IntegratorOutMin=[]  IntegratorOutMax=[]  FilterOutMin=[]  FilterOutMax=[]  SumI1OutMin=[]  SumI1OutMax=[]  SumI2OutMin=[]  SumI2OutMax=[]  SumI3OutMin=[]  SumI3OutMax=[]  SumI4OutMin=[]  SumI4OutMax=[]  SumDOutMin=[]  SumDOutMax=[]  DifferentiatorOutMin=[]  DifferentiatorOutMax=[]  FilterDiffOutCoefMin=[]  FilterDiffOutCoefMax=[]  ReciprocalOutMin=[]  ReciprocalOutMax=[]  SumDenOutMin=[]  SumDenOutMax=[]  SumNumOutMin=[]  SumNumOutMax=[]  DivideOutMin=[]  DivideOutMax=[]  UdiffTsProdOutMin=[]  UdiffTsProdOutMax=[]  NTsProdOutMin=[]  NTsProdOutMax=[]  UintegralTsProdOutMin=[]  UintegralTsProdOutMax=[]  UngainTsProdOutMin=[]  UngainTsProdOutMax=[]  ClampingZeroOutDataTypeStr=Inherit: Inherit via back propagation  ClampingZeroOutMin=[]  ClampingZeroOutMax=[]  FilterDenConstantOutDataTypeStr=Inherit: Inherit via back propagation  FilterDenConstantOutMin=[]  FilterDenConstantOutMax=[]  PCopyOutDataTypeStr=Inherit: Inherit via back propagation  PCopyOutMin=[]  PCopyOutMax=[]  NCopyOutDataTypeStr=Inherit: Inherit via back propagation  NCopyOutMin=[]  NCopyOutMax=[]  IntegratorContinuousStateAttributes=''  IntegratorStateMustResolveToSignalObject=off  IntegratorRTWStateStorageClass=Auto  FilterContinuousStateAttributes=''  FilterStateMustResolveToSignalObject=off  FilterRTWStateStorageClass=Auto  ParallelPVariant=ExternalParameters  IdealPVariant=Disabled  IVariant=ExternalParameters  DVariant=Disabled  IntegratorVariant=Discrete  SatVariant=Enabled  AWVariant=DiscClampingParallel  PCopyVariant=Disabled  TRVariant=Disabled  FdbkBlocksVariant=Forward  IdealPFdbkVariant=Disabled  SatFdbkVariant=Disabled  DerivativeFilterVariant=Disabled  NVariant=Disabled  NCopyVariant=Disabled_SignalSpec  FilterICVariant=Disabled  IntegratorICVariant=ExternalICs  ExternalResetVariant=ExternalReset  TRSumVariant=Passthrough  SumFdbkVariant=Disabled  SumVariant=Sum_PI  TsampFilterVariant=InternalTs  TsampNgainVariant=Passthrough  TsampIntegralVariant=Disabled_SignalSpec  ExternalSaturationOutDataTypeStr=Inherit: Same as second input
      settings: LibrarySourceBlock=mcbcontrolslib/PI Controller
  Ki1 : Constant  Value=PI_params.Ki_speed*Ts_speed  OutDataTypeStr=dataType  SampleTime=-1
  Ki2 : Constant  Value=0  OutDataTypeStr=dataType  SampleTime=-1
  Kp1 : Constant  Value=PI_params.Kp_speed  OutDataTypeStr=dataType  SampleTime=-1
  Logical Operator : Logic  Operator=NOT  IconShape=distinctive  AllPortsSameDT=off  OutDataTypeStr=boolean
  Scope : Scope  NumInputPorts=2
  Sum : Sum  Inputs=|+-  OutDataTypeStr=Inherit: Same as first input
  Iq_ref : Outport  VectorParamsAs1DForOutWhenUnconnected=off
  W_ref : Outport  Port=2  VectorParamsAs1DForOutWhenUnconnected=off
  Speed_meas : Outport  Port=3  VectorParamsAs1DForOutWhenUnconnected=off
  wires:
  Discrete PI Controller with anti-windup & reset/1 -> Iq_ref/1
  Ki1/1 -> Discrete PI Controller with anti-windup & reset/3
  Kp1/1 -> Discrete PI Controller with anti-windup & reset/2
  N_fb/1 -> Scope/2, Speed_meas/1, Sum/2  "SpeedMeas"
  Sum/1 -> Discrete PI Controller with anti-windup & reset/1
  Logical Operator/1 -> Discrete PI Controller with anti-windup & reset/4
  Ki2/1 -> Discrete PI Controller with anti-windup & reset/5
  Data Store Read1/1 -> AND/1
  Data Store Read2/1 -> AND/2
  AND/1 -> Logical Operator/1
  N_ref/1 -> Scope/1, W_ref/1, Sum/1  "SpeedRef"

== system FOCsimulation/FOC/Speed Control/Speed_Ref_Selector ==
  Speed_Ref : Inport
  Absolute value : Subsystem
  Constant : Constant  Value=Speed_openLoop_PU  OutDataTypeStr=dataType
  Constant1 : Constant  Value=-Speed_openLoop_PU  OutDataTypeStr=dataType
  Data Store Read : DataStoreRead  DataStoreName=Speed_ref  IndexOptions=Index vector (dialog)  Indices=1  OutputSizes=1
  Data Store Read1 : DataStoreRead  DataStoreName=EnClosedLoop  IndexOptions=Index vector (dialog)  Indices=1  OutputSizes=1
  Switch : Switch  Criteria=u2 > Threshold  SaturateOnIntegerOverflow=off  InputSameDT=off
  Switch1 : Switch  Criteria=u2 > Threshold  SaturateOnIntegerOverflow=off  InputSameDT=off
  Zero_Cancellation : mcbcontrolslib/IIR Filter  VariantControl=Low Pass Filter  VariantSelect=Low-pass  Filter_constant=0.01*(Ts_speed/Ts)  advancedSettings=off  Ts=50e-6  cutOff_freq=1364.1852
  Speed_Ref1 : Outport
  wires:
  Data Store Read1/1 -> Switch/2
  Constant/1 -> Switch1/1
  Data Store Read/1 -> Switch1/2
  Switch1/1 -> Switch/3
  Constant1/1 -> Switch1/3
  Speed_Ref/1 -> Absolute value/1(Speed_Ref)
  Absolute value/1(Out1) -> Switch/1
  Switch/1 -> Zero_Cancellation/1  "Speed_Ref"
  Zero_Cancellation/1 -> Speed_Ref1/1

== system FOCsimulation/Input/Generated Signal/0.05s // [Ts=2.1s] ==
  Demux : Demux  Tag=STV Demux  Outputs=1
      settings: DisplayOption=none
  FromWs : FromWorkspace  Tag=STV FromWs  VariableName=tuvar
      SigBuilderData=|
      | common.afterFinalStr = 'Extrapolate'
      | common.sampleTime = 0
      | dataSet.timeRange = [0 2.1]
      | dataSet.name = 'Group 1'
      | sbobj.Groups.Name = 'Group 1'
      | sbobj.Groups.Signals.Name = 'Signal 1'
      | sbobj.Groups.Signals.XData = [0 1 1 1.05 1.05 1.1 1.1 1.15 1.15 1.2 1.2 1.25 1.25 1.3 1.3 1.35 1.35 1.4 1.4 1.45 1.45 1.5 1.5 1.55 1.55 1.6 1.6 1.65 1.65 1.7 1.7 1.75 1.75 1.8 1.8 1.85 1.85 1.9 1.9 2.1]
      | sbobj.Groups.Signals.YData = [0.06 0.06 0.1 0.1 0.2 0.2 0.3 0.3 0.4 0.4 0.5 0.5 0.6 0.6 0.7 0.7 0.8 0.8 0.9 0.9 1 1 0.9 0.9 0.8 0.8 0.7 0.7 0.6 0.6 0.5 0.5 0.4 0.4 0.3 0.3 0.2 0.2 0.1 0.1]
      | sbobj.Groups.TimeRange = [0 2.1]
  Signal 1 : Outport  Tag=STV Outport
  wires:
  Demux/1 -> Signal 1/1
  FromWs/1 -> Demux/1

== system FOCsimulation/Input/Generated Signal/0.05s // [Ts=2.2s] ==
  Demux : Demux  Tag=STV Demux  Outputs=1
      settings: DisplayOption=none
  FromWs : FromWorkspace  Tag=STV FromWs  VariableName=tuvar
      SigBuilderData=|
      | common.afterFinalStr = 'Extrapolate'
      | common.sampleTime = 0
      | dataSet.timeRange = [0 2.1]
      | dataSet.name = 'Group 1'
      | sbobj.Groups.Name = 'Group 1'
      | sbobj.Groups.Signals.Name = 'Signal 1'
      | sbobj.Groups.Signals.XData = [0 1 1 1.05 1.05 1.1 1.1 1.15 1.15 1.2 1.2 1.25 1.25 1.3 1.3 1.35 1.35 1.4 1.4 1.45 1.45 1.5 1.5 1.55 1.55 1.6 1.6 1.65 1.65 1.7 1.7 1.75 1.75 1.8 1.8 1.85 1.85 1.9 1.9 1.957 1.957 2.1]
      | sbobj.Groups.Signals.YData = [0.06 0.06 0.1 0.1 0.2 0.2 0.1 0.1 0.4 0.4 0.2 0.2 0.6 0.6 0.3 0.3 0.8 0.8 0.4 0.4 1 1 0.1 0.1 0.9 0.9 0.2 0.2 0.8 0.8 0.3 0.3 0.7 0.7 0.4 0.4 0.6 0.6 0.5 0.5 0.11 0.11]
      | sbobj.Groups.TimeRange = [0 2.1]
  Signal 1 : Outport  Tag=STV Outport
  wires:
  Demux/1 -> Signal 1/1
  FromWs/1 -> Demux/1

== system FOCsimulation/Input/Generated Signal/0.2s // [Ts=4.3s] ==
  Demux : Demux  Tag=STV Demux  Outputs=1
      settings: DisplayOption=none
  FromWs : FromWorkspace  Tag=STV FromWs  VariableName=tuvar
      SigBuilderData=|
      | common.afterFinalStr = 'Extrapolate'
      | common.sampleTime = 0
      | dataSet.timeRange = [0 4.3]
      | dataSet.name = 'Group 1'
      | sbobj.Groups.Name = 'Group 1'
      | sbobj.Groups.Signals.Name = 'Signal 1'
      | sbobj.Groups.Signals.XData = [0 1 1 1.1 1.1 1.3 1.3 1.33 1.33 1.53 1.53 1.56 1.56 1.76 1.76 1.79 1.79 1.99 1.99 2.02 2.02 2.22 2.22 2.42 2.42 2.62 2.62 2.82 2.82 3.02 3.02 3.22 3.22 3.42 3.42 3.62 3.62 3.82 3.82 3.85 3.85 4.05 4.05 4.3]
      | sbobj.Groups.Signals.YData = [0.06 0.06 0.1 0.1 0.2 0.2 0.1 0.1 0.4 0.4 0.1 0.1 0.6 0.6 0.1 0.1 0.8 0.8 0.1 0.1 1 1 0.8 0.8 1 1 0.6 0.6 1 1 0.4 0.4 1 1 0.2 0.2 1 1 0.1 0.1 1 1 0.5 0.5]
      | sbobj.Groups.TimeRange = [0 4.3]
  Signal 1 : Outport  Tag=STV Outport
  wires:
  Demux/1 -> Signal 1/1
  FromWs/1 -> Demux/1

== system FOCsimulation/Input/Generated Signal/0.2s // [Ts=5.3s] ==
  Demux : Demux  Tag=STV Demux  Outputs=1
      settings: DisplayOption=none
  FromWs : FromWorkspace  Tag=STV FromWs  VariableName=tuvar
      SigBuilderData=|
      | common.afterFinalStr = 'Extrapolate'
      | common.sampleTime = 0
      | dataSet.timeRange = [0 5.3]
      | dataSet.name = 'Group 1'
      | sbobj.Groups.Name = 'Group 1'
      | sbobj.Groups.Signals.Name = 'Signal 1'
      | sbobj.Groups.Signals.XData = [0 1 1 1.2 1.2 1.4 1.4 1.6 1.6 1.8 1.8 2 2 2.2 2.2 2.4 2.4 2.6 2.6 2.8 2.8 3 3 3.2 3.2 3.4 3.4 3.6 3.6 3.8 3.8 4 4 4.2 4.2 4.4 4.4 4.6 4.6 4.8 4.8 5 5 5.3]
      | sbobj.Groups.Signals.YData = [0.06 0.06 0.1 0.1 0.2 0.2 0.1 0.1 0.4 0.4 0.1 0.1 0.6 0.6 0.1 0.1 0.8 0.8 0.1 0.1 1 1 0.8 0.8 1 1 0.6 0.6 1 1 0.4 0.4 1 1 0.2 0.2 1 1 0.1 0.1 1 1 0.5 0.5]
      | sbobj.Groups.TimeRange = [0 5.3]
  Signal 1 : Outport  Tag=STV Outport
  wires:
  Demux/1 -> Signal 1/1
  FromWs/1 -> Demux/1

== system FOCsimulation/Input/Generated Signal/0.3s // [Ts=7.5s] ==
  Demux : Demux  Tag=STV Demux  Outputs=1
      settings: DisplayOption=none
  FromWs : FromWorkspace  Tag=STV FromWs  VariableName=tuvar
      SigBuilderData=|
      | common.afterFinalStr = 'Extrapolate'
      | common.sampleTime = 0
      | dataSet.timeRange = [0 7.5]
      | dataSet.name = 'Group 1'
      | sbobj.Groups.Name = 'Group 1'
      | sbobj.Groups.Signals.Name = 'Signal 1'
      | sbobj.Groups.Signals.XData = [0 1 1 1.3 1.3 1.6 1.6 1.9 1.9 2.2 2.2 2.5 2.5 2.8 2.8 3.1 3.1 3.4 3.4 3.7 3.7 4 4 4.3 4.3 4.6 4.6 4.9 4.9 5.2 5.2 5.5 5.5 5.8 5.8 6.1 6.1 6.4 6.4 6.7 6.7 7 7 7.5]
      | sbobj.Groups.Signals.YData = [0.06 0.06 0.1 0.1 0.2 0.2 0.1 0.1 0.4 0.4 0.1 0.1 0.6 0.6 0.1 0.1 0.8 0.8 0.1 0.1 1 1 0.8 0.8 1 1 0.6 0.6 1 1 0.4 0.4 1 1 0.2 0.2 1 1 0.1 0.1 1 1 0.5 0.5]
      | sbobj.Groups.TimeRange = [0 7.5]
  Signal 1 : Outport  Tag=STV Outport
  wires:
  Demux/1 -> Signal 1/1
  FromWs/1 -> Demux/1

== system FOCsimulation/Input/Generated Signal/0.5s // [Ts=12s] ==
  Demux : Demux  Tag=STV Demux  Outputs=1
      settings: DisplayOption=none
  FromWs : FromWorkspace  Tag=STV FromWs  VariableName=tuvar
      SigBuilderData=|
      | common.afterFinalStr = 'Extrapolate'
      | common.sampleTime = 0
      | dataSet.timeRange = [0 12]
      | dataSet.name = 'Group 1'
      | sbobj.Groups.Name = 'Group 1'
      | sbobj.Groups.Signals.Name = 'Signal 1'
      | sbobj.Groups.Signals.XData = [0 1 1 1.5 1.5 2 2 2.5 2.5 3 3 3.5 3.5 4 4 4.5 4.5 5 5 5.5 5.5 6 6 6.5 6.5 7 7 7.5 7.5 8 8 8.5 8.5 9 9 9.5 9.5 10 10 10.5 10.5 11 11 12]
      | sbobj.Groups.Signals.YData = [0.06 0.06 0.1 0.1 0.2 0.2 0.1 0.1 0.4 0.4 0.1 0.1 0.6 0.6 0.1 0.1 0.8 0.8 0.1 0.1 1 1 0.8 0.8 1 1 0.6 0.6 1 1 0.4 0.4 1 1 0.2 0.2 1 1 0.1 0.1 1 1 0.5 0.5]
      | sbobj.Groups.TimeRange = [0 12]
  Signal 1 : Outport  Tag=STV Outport
  wires:
  Demux/1 -> Signal 1/1
  FromWs/1 -> Demux/1

== system FOCsimulation/Input/Generated Signal/2s // [Ts=42s] ==
  Demux : Demux  Tag=STV Demux  Outputs=1
      settings: DisplayOption=none
  FromWs : FromWorkspace  Tag=STV FromWs  VariableName=tuvar
      SigBuilderData=|
      | common.afterFinalStr = 'Extrapolate'
      | common.sampleTime = 0
      | dataSet.timeRange = [0 44]
      | dataSet.name = 'Group 1'
      | sbobj.Groups.Name = 'Group 1'
      | sbobj.Groups.Signals.Name = 'Signal 1'
      | sbobj.Groups.Signals.XData = [0 1 1 3 3 5 5 7 7 9 9 11 11 13 13 15 15 17 17 19 19 21 21 23 23 25 25 27 27 29 29 31 31 33 33 35 35 37 37 39 39 41 41 44]
      | sbobj.Groups.Signals.YData = [0.06 0.06 0.1 0.1 0.2 0.2 0.1 0.1 0.4 0.4 0.1 0.1 0.6 0.6 0.1 0.1 0.8 0.8 0.1 0.1 1 1 0.8 0.8 1 1 0.6 0.6 1 1 0.4 0.4 1 1 0.2 0.2 1 1 0.1 0.1 1 1 0.5 0.5]
      | sbobj.Groups.TimeRange = [0 44]
  Signal 1 : Outport  Tag=STV Outport
  wires:
  Demux/1 -> Signal 1/1
  FromWs/1 -> Demux/1

== system FOCsimulation/Input/Generated Signal/4s // [Ts=50s] ==
  Demux : Demux  Tag=STV Demux  Outputs=1
      settings: DisplayOption=none
  FromWs : FromWorkspace  Tag=STV FromWs  VariableName=tuvar
      SigBuilderData=|
      | common.afterFinalStr = 'Extrapolate'
      | common.sampleTime = 0
      | dataSet.timeRange = [0 50]
      | dataSet.name = 'Group 1'
      | sbobj.Groups.Name = 'Group 1'
      | sbobj.Groups.Signals.Name = 'Signal 1'
      | sbobj.Groups.Signals.XData = [0 0.9 0.9 4.9 4.9 8.9 8.9 12.9 12.9 16.9 16.9 20.9 20.91 24.9 24.91 28.9 28.91 32.9 32.91 36.9 36.91 40.9 40.91 44.9 44.91 50]
      | sbobj.Groups.Signals.YData = [0.06 0.06 0.4 0.4 0.2 0.2 0.6 0.6 0.8 0.8 0.3 0.3 0.2 0.2 0.9 0.9 0.5 0.5 0.7 0.7 0.6 0.6 0.46 0.46 0.7 0.7]
      | sbobj.Groups.TimeRange = [0 50]
  Signal 1 : Outport  Tag=STV Outport
  wires:
  Demux/1 -> Signal 1/1
  FromWs/1 -> Demux/1

== system FOCsimulation/Motor//Inverter Model/Sensor_Measurements/Phase currents + offset1 ==
  Phase currents : Inport
  Add : Sum  Inputs=-+
  Data Store Read : DataStoreRead  DataStoreName=IaOffset  IndexOptions=Index vector (dialog)  Indices=1  OutputSizes=1
  Data Store Read1 : DataStoreRead  DataStoreName=IbOffset  IndexOptions=Index vector (dialog)  Indices=1  OutputSizes=1
  Data Type Conversion : DataTypeConversion  OutDataTypeStr=int32  ConvertRealWorld=Stored Integer (SI)  SaturateOnIntegerOverflow=off  RndMeth=Floor
  Data Type Conversion1 : DataTypeConversion  OutDataTypeStr=dataType  SaturateOnIntegerOverflow=off  RndMeth=Floor
  Data Type Conversion3 : DataTypeConversion  OutDataTypeStr=fixdt(1,32,17)  ConvertRealWorld=Stored Integer (SI)  RndMeth=Simplest  SaturateOnIntegerOverflow=off
  Inverting / Non-inverting Current measurement amplifier : Gain  Gain=inverter.invertingAmp  RndMeth=Simplest  OutDataTypeStr=Inherit: Same as input
  Mux1 : Mux  Inputs=2
  Q17 per unit conversion : ArithShift  BitShiftNumber=-6
  Scope : Scope
  Iab_PU : Outport
  wires:
  Q17 per unit conversion/1 -> Data Type Conversion3/1
  Data Store Read/1 -> Mux1/1
  Add/1 -> Q17 per unit conversion/1
  Data Store Read1/1 -> Mux1/2
  Data Type Conversion3/1 -> Data Type Conversion1/1
  Mux1/1 -> Add/1
  Data Type Conversion1/1 -> Inverting / Non-inverting Current measurement amplifier/1
  Data Type Conversion/1 -> Add/2
  Phase currents/1 -> Scope/1, Data Type Conversion/1
  Inverting / Non-inverting Current measurement amplifier/1 -> Iab_PU/1  "Iab_PU"

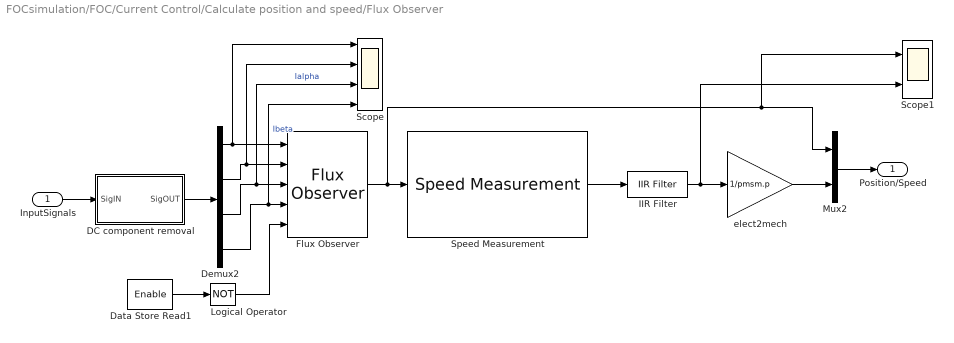
== system FOCsimulation/FOC/Current Control/Calculate position and speed/Flux Observer ==
  InputSignals : Inport
  DC component removal : Subsystem
  Data Store Read1 : DataStoreRead  DataStoreName=Enable  IndexOptions=Index vector (dialog)  Indices=1  OutputSizes=1
  Demux2 : Demux
  Flux Observer : mcbpositiondecoderlib/Flux Observer  MotorSelection=PMSM  DataTypeSelect=off  BlockInputUnit=Per-unit  PerUnitVoltage=PU_System.V_base  PerUnitCurrent=PU_System.I_base  PositionSelect=on  FluxSelect=off  TorqueSelect=off  PolePairs=4  StatorResistance=pmsm.Rs  StatorDAxisInductance=pmsm.Ld  StatorLeakageInductance=0.0068  RotorLeakageInductance=0.0068  MagnetizingInductance=0.0300  CutoffFreq=3.1863  BlockSampleTime=Ts  PositionUnit=Per-unit  PositionDatatype=dataType  FluxUnit=Weber  PerUnitFlux=0.1  FluxDatatype=single  TorqueUnit=Nm  PerUnitTorque=100  TorqueDatatype=single  DataType=0
  IIR Filter : mcbcontrolslib/IIR Filter  VariantControl=Low Pass Filter  VariantSelect=Low-pass  Filter_constant=0.01  advancedSettings=off  Ts=50e-6  cutOff_freq=32.1525
  Logical Operator : Logic  Operator=NOT  IconShape=distinctive  AllPortsSameDT=off  OutDataTypeStr=boolean
  Mux2 : Mux  Inputs=2
  Scope : Scope  NumInputPorts=4
  Scope1 : Scope  NumInputPorts=2
  Speed Measurement : mcbpositiondecoderlib/Speed Measurement  PositionUnit=Per unit  PositionScalingDatatype=uint32  SpeedCalculationMode=Time interval for speed calculation  SampleTimeAsync=Ts  MaximumApplicationSpeed=60000  SpeedResolution=5e-6  DelayLength=10  MaximumMeasurableSpeed=29999  MeasurableSpeedResolution=1.397e-05  SpeedUnit=Per unit based on dialog  PerUnitSpeed=PU_System.N_base  SpeedDataType=dataType
  elect2mech : Gain  Gain=1/pmsm.p  RndMeth=Simplest  OutDataTypeStr=Inherit: Same as input
  Position/Speed : Outport
  wires:
  InputSignals/1 -> DC component removal/1(SigIN)
  Demux2/1 -> Scope/1, Flux Observer/1
  Demux2/2 -> Scope/2, Flux Observer/2
  Mux2/1 -> Position/Speed/1
  Speed Measurement/1 -> IIR Filter/1
  elect2mech/1 -> Mux2/2
  Demux2/3 -> Scope/3, Flux Observer/3  "Ialpha"
  Demux2/4 -> Scope/4, Flux Observer/4  "Ibeta"
  IIR Filter/1 -> Scope1/2, elect2mech/1
  Flux Observer/1 -> Scope1/1, Mux2/1, Speed Measurement/1
  Logical Operator/1 -> Flux Observer/5
  Data Store Read1/1 -> Logical Operator/1
  DC component removal/1(SigOUT) -> Demux2/1

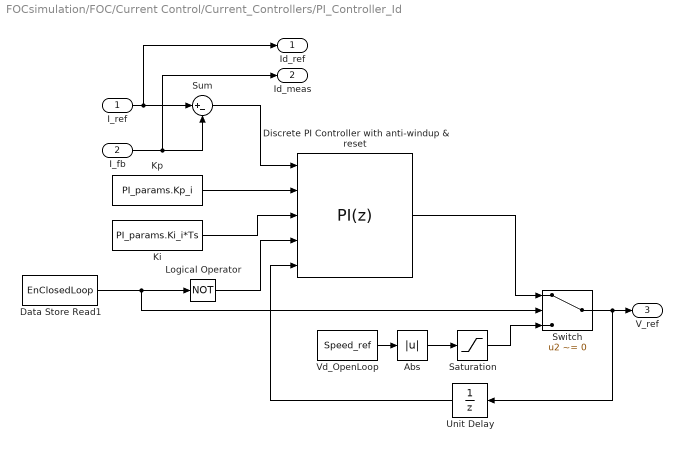
== system FOCsimulation/FOC/Current Control/Current_Controllers/PI_Controller_Id ==
  I_ref : Inport
  I_fb : Inport  Port=2
  Abs : Abs  RndMeth=Simplest  SaturateOnIntegerOverflow=off
  Data Store Read1 : DataStoreRead  DataStoreName=EnClosedLoop  IndexOptions=Index vector (dialog)  Indices=1  OutputSizes=1
  Discrete PI Controller with anti-windup & reset : slpidlib/PID Controller  Controller=PI  Form=Parallel  TimeDomain=Discrete-time  UseExternalTs=off  SampleTime=-1  IntegratorMethod=Forward Euler  FilterMethod=Forward Euler  ControllerParametersSource=external  P=1  I=1  UseKiTs=on  D=0  N=100  UseFilter=on  TunerSelectOption=Transfer Function Based (PID Tuner App)  InitialConditionSource=external  InitialConditionForIntegrator=0  InitialConditionForFilter=0  DifferentiatorICPrevScaledInput=0  ExternalReset=level  TrackingMode=off  Kt=1  LimitOutput=on  SatLimitsSource=internal  UpperSaturationLimit=1  LowerSaturationLimit=-1  LinearizeAsGain=on  AntiWindupMode=clamping  Kb=1  LimitIntegrator=off  UpperIntegratorSaturationLimit=inf  LowerIntegratorSaturationLimit=-inf  RndMeth=Simplest  POutMin=[]  POutMax=[]  IOutMin=[]  IOutMax=[]  DOutMin=[]  DOutMax=[]  NOutMin=[]  NOutMax=[]  SumOutMin=[]  SumOutMax=[]  SaturationOutDataTypeStr=Inherit: Inherit via back propagation  SaturationOutMin=[]  SaturationOutMax=[]  PParamMin=[]  PParamMax=[]  IParamMin=[]  IParamMax=[]  DParamMin=[]  DParamMax=[]  NParamMin=[]  NParamMax=[]  KbParamMin=[]  KbParamMax=[]  KtParamMin=[]  KtParamMax=[]  KbOutMin=[]  KbOutMax=[]  KtOutMin=[]  KtOutMax=[]  IntegratorOutMin=[]  IntegratorOutMax=[]  FilterOutMin=[]  FilterOutMax=[]  SumI1OutMin=[]  SumI1OutMax=[]  SumI2OutMin=[]  SumI2OutMax=[]  SumI3OutMin=[]  SumI3OutMax=[]  SumI4OutMin=[]  SumI4OutMax=[]  SumDOutMin=[]  SumDOutMax=[]  DifferentiatorOutMin=[]  DifferentiatorOutMax=[]  FilterDiffOutCoefMin=[]  FilterDiffOutCoefMax=[]  ReciprocalOutMin=[]  ReciprocalOutMax=[]  SumDenOutMin=[]  SumDenOutMax=[]  SumNumOutMin=[]  SumNumOutMax=[]  DivideOutMin=[]  DivideOutMax=[]  UdiffTsProdOutMin=[]  UdiffTsProdOutMax=[]  NTsProdOutMin=[]  NTsProdOutMax=[]  UintegralTsProdOutMin=[]  UintegralTsProdOutMax=[]  UngainTsProdOutMin=[]  UngainTsProdOutMax=[]  ClampingZeroOutDataTypeStr=Inherit: Inherit via back propagation  ClampingZeroOutMin=[]  ClampingZeroOutMax=[]  FilterDenConstantOutDataTypeStr=Inherit: Inherit via back propagation  FilterDenConstantOutMin=[]  FilterDenConstantOutMax=[]  PCopyOutDataTypeStr=Inherit: Inherit via back propagation  PCopyOutMin=[]  PCopyOutMax=[]  NCopyOutDataTypeStr=Inherit: Inherit via back propagation  NCopyOutMin=[]  NCopyOutMax=[]  IntegratorContinuousStateAttributes=''  IntegratorStateMustResolveToSignalObject=off  IntegratorRTWStateStorageClass=Auto  FilterContinuousStateAttributes=''  FilterStateMustResolveToSignalObject=off  FilterRTWStateStorageClass=Auto  ParallelPVariant=ExternalParameters  IdealPVariant=Disabled  IVariant=ExternalParameters  DVariant=Disabled  IntegratorVariant=Discrete  SatVariant=Enabled  AWVariant=DiscClampingParallel  PCopyVariant=Disabled  TRVariant=Disabled  FdbkBlocksVariant=Forward  IdealPFdbkVariant=Disabled  SatFdbkVariant=Disabled  DerivativeFilterVariant=Disabled  NVariant=Disabled  NCopyVariant=Disabled_SignalSpec  FilterICVariant=Disabled  IntegratorICVariant=ExternalICs  ExternalResetVariant=ExternalReset  TRSumVariant=Passthrough  SumFdbkVariant=Disabled  SumVariant=Sum_PI  TsampFilterVariant=InternalTs  TsampNgainVariant=Passthrough  TsampIntegralVariant=Disabled_SignalSpec  ExternalSaturationOutDataTypeStr=Inherit: Same as second input
      settings: LibrarySourceBlock=mcbcontrolslib/PI Controller
  Ki : Constant  Value=PI_params.Ki_i*Ts  OutDataTypeStr=dataType  SampleTime=-1
  Kp : Constant  Value=PI_params.Kp_i  OutDataTypeStr=dataType  SampleTime=-1
  Logical Operator : Logic  Operator=NOT  IconShape=distinctive  AllPortsSameDT=off  OutDataTypeStr=boolean
  Saturation : Saturate  LowerLimit=0.15  RndMeth=Simplest
  Sum : Sum  Inputs=|+-  OutDataTypeStr=Inherit: Same as first input
  Switch : Switch  Criteria=u2 ~= 0  RndMeth=Simplest  SaturateOnIntegerOverflow=off  InputSameDT=off
  Unit Delay : UnitDelay  SampleTime=-1  HasFrameUpgradeWarning=on
  Vd_OpenLoop : DataStoreRead  DataStoreName=Speed_ref  IndexOptions=Index vector (dialog)  Indices=1  OutputSizes=1
  Id_ref : Outport  VectorParamsAs1DForOutWhenUnconnected=off
  Id_meas : Outport  Port=2  VectorParamsAs1DForOutWhenUnconnected=off
  V_ref : Outport  Port=3  VectorParamsAs1DForOutWhenUnconnected=off
  wires:
  Switch/1 -> V_ref/1, Unit Delay/1
  I_fb/1 -> Id_meas/1, Sum/2
  Sum/1 -> Discrete PI Controller with anti-windup & reset/1
  Kp/1 -> Discrete PI Controller with anti-windup & reset/2
  I_ref/1 -> Id_ref/1, Sum/1
  Ki/1 -> Discrete PI Controller with anti-windup & reset/3
  Logical Operator/1 -> Discrete PI Controller with anti-windup & reset/4
  Unit Delay/1 -> Discrete PI Controller with anti-windup & reset/5
  Discrete PI Controller with anti-windup & reset/1 -> Switch/1
  Data Store Read1/1 -> Logical Operator/1, Switch/2
  Saturation/1 -> Switch/3
  Abs/1 -> Saturation/1
  Vd_OpenLoop/1 -> Abs/1
